simulink model "PassVeh14DOF"  (R2026b)
settings: Solver=ode23tb  StopTime=inf  FixedStep=.001  RelTol=1e-1  EnableMultiTasking=on
model workspace (MAT data in the model file):
  AlgnTrqCambCompl = [0 0 0 0]
  AlgnTrqSteerCompl = [0 0 0 0]
  AxlIxx = 62.3745166667
  AxlM = 160
  BumpCamber = [0 0 0 0]
  BumpCaster = [0 0 0 0]
  BumpSteer = [0 0 0 0]
  CambVsSteerAng = [0 0 0 0]
  CastVsSteerAng = [0 0 0 0]
  Cps = 2
  Cz = 5565.2246438
  CzWhlAxl = 11490.971257
  DCT_Param : object (value not decoded)
  Downshift_Speeds = [9.5625 12.9375 16.3125 19.6875 23.0625 26.4375 29.8125 33.1875 36.5625 39.9375 43.3125 46.6875 ... (28 elements, 4x7)]
  F0z = [2886 2907]
  F0zWhlAxl = 2907
  Hmax = 0.25
  Kz = 52451.0065793
  KzWhlAxl = 138031.612078
  LatCambCompl = [0 0 0 0]
  LatSteerCompl = [0 0 0 0]
  LatWhlCtrComplLat = [0 0 0 0]
  LatWhlCtrComplLng = [0  0  0  0; 0  0  0  0]
  LatWhlCtrDisp = [0 0 0 0]
  LngCambCompl = [0  0  0  0; 0  0  0  0]
  LngCastCompl = [0  0  0  0; 0  0  0  0]
  LngSteerCompl = [0  0  0  0; 0  0  0  0]
  LngWhlCtrCompl = [0  0  0  0; 0  0  0  0]
  LngWhlCtrDisp = [0 0 0 0]
  MotRatios = [1 1]
  NCyl = 6
  NrmlWhlFrcOff = [2886 2886 2907 2907]
  NrmlWhlRates = [52.4510065793 52.4510065793 52.4510065793 52.4510065793]
  Pedal_Positions = [0.1 0.4 0.5 0.9]
  Pstd = 101325
  Rair = 287
  RollCamber : object (value not decoded)
  RollCaster : object (value not decoded)
  RollSteer : object (value not decoded)
  RollStiffArb = [0 0]
  RollStiffArbFrnt = 800
  RollStiffNoArb = [0 0]
  RollStiffNoArbFrnt = 0
  RollStiffNoTwstRear = 0
  ShckFrcVsCompRate = [5.5652246438 5.5652246438 5.5652246438 5.5652246438]
  StatCamber = [0 0 0 0]
  StatCaster = [0 0 0 0]
  StatLdWhlR = [0.3 0.3 0.3 0.3]
  StatToe = [0 0 0 0]
  Trans : object (value not decoded)
  Tstd = 293.15
  Upshift_Speeds = [12.9375 16.3125 19.6875 33 26.4375 29.8125 33.1875 52.5 39.9375 43.3125 46.6875 77.25 ... (28 elements, 4x7)]
  VEH : object (value not decoded)
  Vd = 0.00346
  VrtLdTrnsfr = [0 0 0 0]
  WH : Mass (value not decoded)
  dt3D = 0.05
  f_air = [0 0 0 0 0 0 0 0 0 0 0 0 ... (256 elements, 16x16)]
  f_co = [0 0 0 0 0 0 0 0 0 0 0 0 ... (256 elements, 16x16)]
  f_co2 = [0 0 0 0 0 0 0 0 0 0 0 0 ... (256 elements, 16x16)]
  f_eff = [352.135682859 352.135682859 320.724378192 303.655312657 295.930136708 291.240087194 291.240271258 291.240312459 291.240275452 291.240198499 291.240100781 291.240018769 ... (256 elements, 16x16)]
  f_fuel = [0 0 0 0 0 0 0 0 0 0 0 0 ... (256 elements, 16x16)]
  f_hc = [0 0 0 0 0 0 0 0 0 0 0 0 ... (256 elements, 16x16)]
  f_nox = [0 0 0 0 0 0 0 0 0 0 0 0 ... (256 elements, 16x16)]
  f_pm = [0 0 0 0 0 0 0 0 0 0 0 0 ... (256 elements, 16x16)]
  f_susp_axl_bp = [1 2]
  f_susp_dz_bp = [-0.325022776267 -0.315022776267 -0.305022776267 -0.205022776267 -0.105022776267 -0.00502277626717 0.0949772237328 0.194977223733 0.204977223733 0.214977223733]
  f_susp_dzdot_bp = [-3 -0.3 -0.2 -0.1 0 0.1 0.2 0.3 3]
  f_susp_fmz = [-144070.391448 -93629.24037 -75929.1118915 -20630.5828179 -15385.48216 -10140.3815021 -4895.28084414 349.819813785 -31916.3973792 18437.6709544 -83996.1993354 -33555.0482577 ... (43920 elements, 10x9x61x2x4)]
  f_susp_geom = [0 0 0 0 0 0 0 0 0 0 0 0 ... (3660 elements, 10x61x2x3)]
  f_susp_strgdelta_bp = [-0.523598775598 -0.506145483078 -0.488692190558 -0.471238898038 -0.453785605519 -0.436332312999 -0.418879020479 -0.401425727959 -0.383972435439 -0.366519142919 -0.349065850399 -0.331612557879 ... (61 elements, 1x61)]
  f_tbrake = [0 76.8593923996 105.140482948 131.533638111 157.926793274 176.658631717 176.65727296 176.656856686 176.656879077 176.657093756 176.657404516 176.65772406 ... (256 elements, 16x16)]
  f_tbrake_n_bpt = [0 649.519052838 912.419621844 1175.32019085 1438.22075986 1701.12132886 1964.02189787 2226.92246687 2489.82303588 2752.72360489 3015.62417389 3278.5247429 ... (16 elements, 1x16)]
  f_tbrake_t_bpt = [0 34.6410161514 61.0341713143 87.4273264773 113.82048164 140.213636803 166.606791966 192.999947129 219.393102292 245.786257455 272.179412618 298.572567781 ... (16 elements, 1x16)]
  f_texh = [766.752464599 766.752464599 786.17542386 801.679939032 884.591982581 910.574397722 910.571871054 910.570774534 910.570601632 910.570821151 910.571247242 910.571639815 ... (256 elements, 16x16)]
  f_twc_eff_co = [0.17 0.25 0.45 0.99 0.99 0.99 0.99]
  f_twc_eff_hc = [0.21 0.375 0.75 0.98 0.98 0.98 0.98]
  f_twc_eff_lam = [0.909090909 0.944055944 0.979020979 1 1.013986014 1.048951049 1.083916084]
  f_twc_eff_nox = [0.98 0.98 0.98 0.97 0.05 0.02 0]
  numWheel = 4
symbols that are objects in the model workspace (value not decoded): VEH
libraries: vehdynlibtire x12, vehdynlibsuspension x8, autolibutils x5, sharedtransform x5, shared6dof x2, vehdynlibeom x1, vehdynlibtirecommon x1, matrix_library x1
(part 8 of 9)

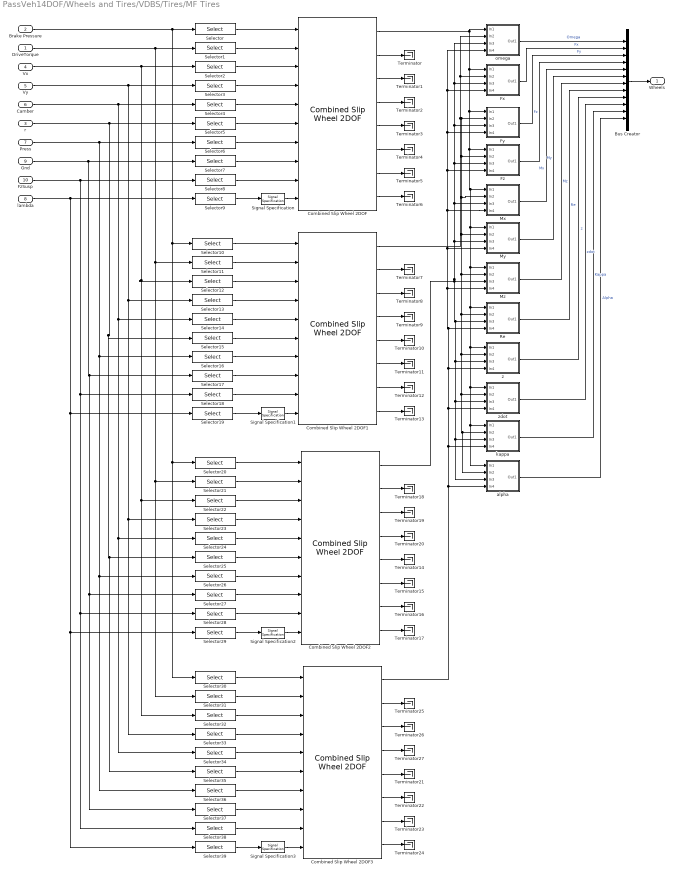
== system PassVeh14DOF/Wheels and Tires/VDBS/Tires/MF Tires ==
  DriveTorque : Inport
  Brake Pressure : Inport  Port=2
  r : Inport  Port=3
  Vx : Inport  Port=4
  Vy : Inport  Port=5
  Camber : Inport  Port=6
  Press : Inport  Port=7  Unit=Pa
  lambda : Inport  Port=8  Unit=1
  Gnd : Inport  Port=9
  FzSusp : Inport  Port=10
  Bus Creator : BusCreator  Inputs=12
  Combined Slip Wheel 2DOF{,1..3} (4 alike) : vehdynlibtire/Combined Slip Wheel 2DOF  tireType=Mid-size passenger car 235/45R18  tireParamSet=vdynPassCar.mat  scaleFactorInput=on  vertType=Magic Formula  plySteer=off  turnslip=off  BrakeType=Disc  mu_static=.3  mu_kinetic=.2  drum_abore=0.0508  drum_a=0.123  drum_c=0.212  drum_r=0.15  drum_theta1=0  drum_theta2=126  disk_abore=.05  Rm=.177  num_pads=2  brake_p_bpt=[1 11.4736842105263 21.9473684210526 32.4210526315789 42.8947368421053 53.3684210526316 63.8421052631579 74.3157894736842 84.7894736842105 95.2631578947368 105.736842105263 116.210526315789 126.684210526316 137.157894736842 147.631578947368 158.105263157895 168.578947368421 179.052631578947 189.526315789474 200]  brake_n_bpt=[0 52.6315789473684 105.263157894737 157.894736842105 210.526315789474 263.157894736842 315.789473684211 368.421052631579 421.052631578947 473.684210526316 526.315789473684 578.947368421053 631.578947368421 684.210526315789 736.842105263158 789.473684210526 842.105263157895 894.736842105263 947.368421052632 1000]  f_brake_t=[43.4900602404453 42.5056030554862 41.5350898940194 40.5780454442085 39.6340111501808 38.7025443887544 37.7832176914519 36.8756180088306 35.9793460143796 35.0940154454303 34.2192524787115 33.3546951383474 32.4999927342521 31.6548053290159 30.8188032315107 29.991666515561 29.1730845621415 28.362755623661 27.5603864089927 26.765691687993;498.991217495636 487.695866636631 476.560505099801 465.579679307235 454.748127933653 444.060772460445 433.51270824929 423.099196101319 412.81565427025 402.657650900201 392.620896861006 382.701238955775 372.894653477208 363.197240090814 353.605216024701 344.114910546964 334.722759712992 325.425301366216 316.219170376863 307.10109410434;954.492374750826 932.886130217776 911.585920305583 890.581313170261 869.862244717126 849.419000532136 829.242198807128 809.322774193808 789.651962526121 770.221286354971 751.0225412433 732.047782773203 713.289314220164 694.739674852612 676.391628817892 658.238154578366 640.272434863842 622.48784710877 604.877954344734 587.436496520688;1409.99353200602 1378.07639379892 1346.61133551136 1315.58294703329 1284.9763615006 1254.77722860383 1224.97168936497 1195.5463522863 1166.48827078199 1137.78492180974 1109.42418562559 1081.39432659063 1053.68397496312 1026.28210961441 999.178041611083 972.361398609768 945.822110014692 919.550392851325 893.536738312604 867.771898937035;1865.49468926121 1823.26665738007 1781.63675071715 1740.58458089631 1700.09047828407 1660.13545667552 1620.7011799228 1581.76993037878 1543.32457903786 1505.34855726451 1467.82583000789 1430.74087040806 1394.07863570608 1357.82454437621 1321.96445440427 1286.48464264117 1251.37178516554 1216.61293859388 1182.19552228048 1148.10730135338;2320.9958465164 2268.45692096121 2216.66216592293 2165.58621475934 2115.20459506754 2065.49368474721 2016.43067048064 1967.99350847127 1920.16088729373 1872.91219271928 1826.22747439018 1780.08741422549 1734.47329644903 1689.36697913801 1644.75086719747 1600.60788667257 1556.92146031639 1513.67548433643 1470.85430624835 1428.44270376973;2776.49700377159 2713.64718454235 2651.68758112871 2590.58784862237 2530.31871185102 2470.8519128189 2412.16016103848 2354.21708656376 2296.9971955496 2240.47582817405 2184.62911877248 2129.43395804292 2074.86795719199 2020.9094138998 1967.53727999066 1914.73113070398 1862.47113546724 1810.73803007899 1759.51309021622 1708.77810618608;3231.99816102678 3158.8374481235 3086.71299633449 3015.58948248539 2945.43282863449 2876.21014089059 2807.88965159632 2740.44066465625 2673.83350380547 2608.03946362882 2543.03076315477 2478.78050186034 2415.26261793494 2352.4518486616 2290.32369278385 2228.85437473538 2168.02081061809 2107.80057582154 2048.17187418409 1989.11350860242;3687.49931828197 3604.02771170464 3521.73841154027 3440.59111634842 3360.54694541796 3281.56836896228 3203.61914215416 3126.66424274874 3050.66981206134 2975.60309908359 2901.43240753707 2828.12704567777 2755.6572786779 2683.9942834234 2613.11010557704 2542.97761876678 2473.57048576894 2404.8631215641 2336.83065815196 2269.44891101877;4143.00047553716 4049.21797528579 3956.76382674606 3865.59275021144 3775.66106220143 3686.92659703397 3599.34863271199 3512.88782084123 3427.50612031721 3343.16673453836 3259.83405191936 3177.4735894952 3096.05193942085 3015.5367181852 2935.89651837023 2857.10086279818 2779.12016091979 2701.92566730665 2625.48944211983 2549.78431343512;4598.50163279235 4494.40823886693 4391.78924195184 4290.59438407447 4190.77517898491 4092.28482510566 3995.07812326983 3899.11139893372 3804.34242857308 3710.73036999313 3618.23569630166 3526.82013331263 3436.44660016381 3347.079152947 3258.68293116342 3171.22410682959 3084.66983607064 2998.98821304921 2914.1482260877 2830.11971585147;5054.00279004754 4939.59850244808 4826.81465715762 4715.59601793749 4605.88929576838 4497.64305317735 4390.80761382767 4285.3349770262 4181.17873682896 4078.2940054479 3976.63734068395 3876.16667713006 3776.84126090677 3678.62158770879 3581.46934395661 3485.34735086099 ...(+2764 chars)]  NOMPRES=262000  PRESMAX=1000000  PRESMIN=10000  FNOMIN=4300  FZMAX=8600  FZMIN=100  VXLOW=1  KPUMAX=1.5  KPUMIN=-1.5  ALPMAX=1.5  ALPMIN=-1.5  CAMMAX=0.17453  CAMMIN=-0.17453  LONGVL=16.7  FxRelFreqLwrLim=200*pi  FyRelFreqLwrLim=0  MyRelFreqLwrLim=50*pi  omegao=0  UNLOADED_RADIUS=0.33454  WIDTH=0.235  RIM_RADIUS=0.2286  ASPECT_RATIO=0.45  MASS=11.2  IYY=1.084  br=1e-3  GRAVITY=-9.81  LFZO=1  LMUX=1  LMUY=1  LMUV=0  LKX=1  LKY=1  LCX=1  LCY=1  LEX=1  LEY=1  LHX=1  LHY=1  LVX=1  LVY=1  LKYC=1  LKZC=1  LTR=1  LRES=1  LXAL=1  LYKA=1  LVYKA=1  LS=1  LCZ=1  LMX=1  LVMX=1  LMY=1  LMP=1  zo=.015+VEH.InitialVertPosition  zdoto=0  BREFF=8.25094594147963  DREFF=0.260468730454265  FREFF=0.0735298544471851  Q_RE0=1.00866439868088  Q_V1=0.000760413786224011  Q_V2=0.0463384792019201  Q_FZ1=0  Q_FZ2=15.6870832810226  Q_FZ3=0  Q_FCX=0.138643970247602  Q_FCY=0.10843499565426  Q_FCY2=-0.465763352339538  PFZ1=0.69958166705601  VERTICAL_STIFFNESS=207885.061134007  VERTICAL_DAMPING=500  BOTTOM_OFFST=0.00990653336182505  BOTTOM_STIFF=1999075.87051971  Q_CAM1=0  Q_CAM2=0  Q_CAM3=0  Q_FYS1=0  Q_FYS2=0  Q_FYS3=0  LONGITUDINAL_STIFFNESS=388714.175879854  LATERAL_STIFFNESS=157087.404633332  PCFX1=0.18539229191199  PCFX2=0  PCFX3=0  PCFY1=0.163183345037677  PCFY2=0  PCFY3=0.249094918231954  Q_RA1=0.675942571700787  Q_RA2=0.73800463546164  Q_RB1=1.04487486456705  Q_RB2=-1.191763806629  PCX1=1.58523057950359  PDX1=1.0239116238178  PDX2=-0.0842405110022724  PDX3=0  PEX1=0.110312777158455  PEX2=0.313468516038146  PEX3=0  PEX4=0.0016060905760045  PKX1=21.3872544684023  PKX2=14.0006541873175  PKX3=-0.405326109653452  PHX1=0.000212599305364818  PHX2=0.00115950515263055  PVX1=1.59236164471432e-05  PVX2=0.000104321112127671  PPX1=-0.349461321276586  PPX2=0.387840040616429  PPX3=-0.0969947336569324  PPX4=0.0632271859795801  RBX1=12.7633329850276  RBX2=9.5787123658471  RBX3=0  RCX1=1.02796280922059  REX1=-0.45202516851367  REX2=-0.47304886171176  RHX1=0.000233272373115809  QSX1=-0.00788307788961443  QSX2=0.954629515459396  QSX3=0.0155855777667025  QSX4=0.125904607142414  QSX5=1.01110069703963  QSX6=20.1938577118433  QSX7=0.310818120717083  QSX8=-0.0430823751139655  QSX9=0.636494404888216  QSX10=0.142438060591663  QSX11=0.346766530036373  QSX12=0  QSX13=0  QSX14=0  PPMX1=0  PCY1=1.34299950037631  PDY1=0.878267729082195  PDY2=-0.0644597923147385  PDY3=0  PEY1=-0.809776534470972  PEY2=-0.600180598867198  PEY3=0.0991732552633487  PEY4=-6.5577974035573  PEY5=0  PKY1=-15.5714726518315  PKY2=1.73126522291751  PKY3=0.365349873517229  PKY4=1.98176755955416  PKY5=0  PKY6=-0.884005199550313  PKY7=-0.237259727611847  PHY1=-0.00183370557235628  PHY2=0.00346401302716671  PVY1=-0.00675427560163264  PVY2=0.036379218103843  PVY3=-0.163543984089166  PVY4=-0.491003349625726  PPY1=-0.62059646553185  PPY2=-0.0647824842338686  PPY3=-0.164648843290686  PPY4=0.283193909060098  PPY5=0  RBY1=10.7588809173639  RBY2=7.70420065295029  RBY3=3.40283755070691e-06  RBY4=0  RCY1=1.06691874059059  REY1=0.308244924574305  REY2=7.48775032604508e-06  RHY1=0.0118479204960415  RHY2=7.63650177161071e-06  RVY1=0.0560024425050078  RVY2=7.48487127056197e-06  RVY3=0  RVY4=98.4047026517149  RVY5=2.02759273900054  RVY6=15.7623064923347  QSY1=0.00699077564863536  QSY2=0  QSY3=0.00153535478298811  QSY4=8.55710322455322e-05  QSY5=0  QSY6=0  QSY7=0.89443879773793  QSY8=-0.403227641260894  QBZ1=11.666656027484  QBZ2=-1.30355438574485  QBZ3=0  QBZ4=0.177918305399071  QBZ5=-0.162481135068033  QBZ6=0  QBZ9=30.1445534682089  QBZ10=0  QCZ1=1.29026978207574  QDZ1=0.0886972644991399  QDZ2=-0.0058634820161856  QDZ3=0.3805597481383  QDZ4=0  QDZ6=0.00160914918118959  QDZ7=-0.00211036330862154  QDZ8=-0.13921904912557  QDZ9=0.00816585550028243  QDZ10=0  QDZ11=0  QEZ1=-2.19802254534746  QEZ2=1.01850535789165  QEZ3=0  QEZ4=0.278379679112054  QEZ5=-0.548414722765386  QHZ1=0.00148361198869669  QHZ2=0.00202017567585904  QHZ3=0.240316641332066  QHZ4=-0.210114035738085  PPZ1=-0.443927982388615  PPZ2=0  SSZ1=0.00914999585397887  SSZ2=0.0389830656052735  SSZ3=0  SSZ4=0  PDXP1=0.396718274678791  PDXP2=0  PDXP3=0  PKYP1=1.00587060633573  PDYP1=0.40483048923438  PDYP2=0  PDYP3=0  PDYP4=0  PHYP1=0.992731942067188  PHYP2=0.150352945499914  PHYP3=0  PHYP4=-3.98988682633674  PECP1=0.502379254513503  PECP2=0  QDTP1=10.0178654287947  QCRP1=0.200627747200702  QCRP2=0.0995735881599772  QBRP1=0.0997107127960717  QDRP1=1.01432910167423  QDRP2=0  aMode=2
  Fx : Subsystem
  Fy : Subsystem
  Fz : Subsystem
  Mx : Subsystem
  My : Subsystem
  Mz : Subsystem
  Re : Subsystem
  Selector{,1..8} (9 alike) : Selector  InputPortWidth=4  IndexOptions=Index vector (dialog)  Indices=1  OutputSizes=1
  Selector{10..18} (9 alike) : Selector  InputPortWidth=4  IndexOptions=Index vector (dialog)  Indices=2  OutputSizes=1
  Selector19 : Selector  NumberOfDimensions=2  InputPortWidth=4  IndexOptions=Select all,Index vector (dialog)  Indices=1,2  OutputSizes=1,1
  Selector{20..28} (9 alike) : Selector  InputPortWidth=4  IndexOptions=Index vector (dialog)  Indices=3  OutputSizes=1
  Selector29 : Selector  NumberOfDimensions=2  InputPortWidth=4  IndexOptions=Select all,Index vector (dialog)  Indices=1,3  OutputSizes=1,1
  Selector{30..38} (9 alike) : Selector  InputPortWidth=4  IndexOptions=Index vector (dialog)  Indices=4  OutputSizes=1
  Selector39 : Selector  NumberOfDimensions=2  InputPortWidth=4  IndexOptions=Select all,Index vector (dialog)  Indices=1,4  OutputSizes=1,1
  Selector9 : Selector  NumberOfDimensions=2  InputPortWidth=4  IndexOptions=Select all,Index vector (dialog)  Indices=1,1  OutputSizes=1,1
  Signal Specification{,1..3} (4 alike) : SignalSpecification  Unit=1
  Terminator{,1..27} (28 alike) : Terminator
  alpha : Subsystem
  kappa : Subsystem
  omega : Subsystem
  z : Subsystem
  zdot : Subsystem
  Wheels : Outport  VectorParamsAs1DForOutWhenUnconnected=off
  wires:
  Bus Creator/1 -> Wheels/1
  Brake Pressure/1 -> Selector30/1, Selector20/1, Selector10/1, Selector/1
  DriveTorque/1 -> Selector31/1, Selector21/1, Selector11/1, Selector1/1
  Vx/1 -> Selector12/1, Selector32/1, Selector22/1, Selector2/1
  Selector/1 -> Combined Slip Wheel 2DOF/1
  Selector1/1 -> Combined Slip Wheel 2DOF/2
  Selector7/1 -> Combined Slip Wheel 2DOF/8
  Selector6/1 -> Combined Slip Wheel 2DOF/7
  Selector5/1 -> Combined Slip Wheel 2DOF/6
  Selector4/1 -> Combined Slip Wheel 2DOF/5
  Selector9/1 -> Signal Specification/1
  Selector8/1 -> Combined Slip Wheel 2DOF/9
  Camber/1 -> Selector34/1, Selector24/1, Selector14/1, Selector4/1
  Vy/1 -> Selector33/1, Selector23/1, Selector13/1, Selector3/1
  r/1 -> Selector15/1, Selector35/1, Selector25/1, Selector5/1
  Press/1 -> Selector36/1, Selector26/1, Selector16/1, Selector6/1
  Gnd/1 -> Selector37/1, Selector27/1, Selector17/1, Selector7/1
  FzSusp/1 -> Selector38/1, Selector28/1, Selector18/1, Selector8/1
  lambda/1 -> Selector9/1, Selector19/1, Selector39/1, Selector29/1
  Selector18/1 -> Combined Slip Wheel 2DOF1/9
  Selector19/1 -> Signal Specification1/1
  Selector14/1 -> Combined Slip Wheel 2DOF1/5
  Selector15/1 -> Combined Slip Wheel 2DOF1/6
  Selector16/1 -> Combined Slip Wheel 2DOF1/7
  Selector17/1 -> Combined Slip Wheel 2DOF1/8
  Selector12/1 -> Combined Slip Wheel 2DOF1/3
  Selector13/1 -> Combined Slip Wheel 2DOF1/4
  Selector11/1 -> Combined Slip Wheel 2DOF1/2
  Selector10/1 -> Combined Slip Wheel 2DOF1/1
  Selector30/1 -> Combined Slip Wheel 2DOF3/1
  Selector31/1 -> Combined Slip Wheel 2DOF3/2
  Selector33/1 -> Combined Slip Wheel 2DOF3/4
  Selector32/1 -> Combined Slip Wheel 2DOF3/3
  Selector37/1 -> Combined Slip Wheel 2DOF3/8
  Selector36/1 -> Combined Slip Wheel 2DOF3/7
  Selector35/1 -> Combined Slip Wheel 2DOF3/6
  Selector34/1 -> Combined Slip Wheel 2DOF3/5
  Selector39/1 -> Signal Specification3/1
  Selector38/1 -> Combined Slip Wheel 2DOF3/9
  Selector28/1 -> Combined Slip Wheel 2DOF2/9
  Selector29/1 -> Signal Specification2/1
  Selector24/1 -> Combined Slip Wheel 2DOF2/5
  Selector25/1 -> Combined Slip Wheel 2DOF2/6
  Selector26/1 -> Combined Slip Wheel 2DOF2/7
  Selector27/1 -> Combined Slip Wheel 2DOF2/8
  Selector22/1 -> Combined Slip Wheel 2DOF2/3
  Selector23/1 -> Combined Slip Wheel 2DOF2/4
  Selector21/1 -> Combined Slip Wheel 2DOF2/2
  Selector20/1 -> Combined Slip Wheel 2DOF2/1
  Combined Slip Wheel 2DOF1/1 -> omega/2(In2), Fx/2(In2), Mx/2(In2), My/2(In2), alpha/2(In2), kappa/2(In2), zdot/2(In2), z/2(In2), Re/2(In2), Mz/2(In2), Fz/2(In2), Fy/2(In2)
  Combined Slip Wheel 2DOF2/1 -> omega/3(In3), Fx/3(In3), Fy/3(In3), Fz/3(In3), Mx/3(In3), My/3(In3), alpha/3(In3), kappa/3(In3), zdot/3(In3), z/3(In3), Re/3(In3), Mz/3(In3)
  Combined Slip Wheel 2DOF3/1 -> omega/4(In4), Fx/4(In4), Fy/4(In4), Fz/4(In4), Mx/4(In4), My/4(In4), Mz/4(In4), Re/4(In4), z/4(In4), zdot/4(In4), kappa/4(In4), alpha/4(In4)
  Combined Slip Wheel 2DOF/1 -> omega/1(In1), Mx/1(In1), My/1(In1), alpha/1(In1), kappa/1(In1), zdot/1(In1), z/1(In1), Re/1(In1), Mz/1(In1), Fz/1(In1), Fy/1(In1), Fx/1(In1)
  omega/1(Out1) -> Bus Creator/1  "Omega"
  Fx/1(Out1) -> Bus Creator/2  "Fx"
  Mz/1(Out1) -> Bus Creator/7  "Mz"
  Fz/1(Out1) -> Bus Creator/4  "Fz"
  Re/1(Out1) -> Bus Creator/8  "Re"
  z/1(Out1) -> Bus Creator/9  "z"
  zdot/1(Out1) -> Bus Creator/10  "zdot"
  Mx/1(Out1) -> Bus Creator/5  "Mx"
  My/1(Out1) -> Bus Creator/6  "My"
  kappa/1(Out1) -> Bus Creator/11  "Kappa"
  Fy/1(Out1) -> Bus Creator/3  "Fy"
  Selector2/1 -> Combined Slip Wheel 2DOF/3
  Selector3/1 -> Combined Slip Wheel 2DOF/4
  Signal Specification/1 -> Combined Slip Wheel 2DOF/10
  Signal Specification1/1 -> Combined Slip Wheel 2DOF1/10
  Signal Specification2/1 -> Combined Slip Wheel 2DOF2/10
  Signal Specification3/1 -> Combined Slip Wheel 2DOF3/10
  Combined Slip Wheel 2DOF/2 -> Terminator/1
  Combined Slip Wheel 2DOF/3 -> Terminator1/1
  Combined Slip Wheel 2DOF/4 -> Terminator2/1
  Combined Slip Wheel 2DOF/7 -> Terminator5/1
  Combined Slip Wheel 2DOF/6 -> Terminator4/1
  Combined Slip Wheel 2DOF/5 -> Terminator3/1
  Combined Slip Wheel 2DOF/8 -> Terminator6/1
  Combined Slip Wheel 2DOF1/2 -> Terminator7/1
  Combined Slip Wheel 2DOF1/3 -> Terminator8/1
  Combined Slip Wheel 2DOF1/4 -> Terminator9/1
  Combined Slip Wheel 2DOF1/5 -> Terminator10/1
  Combined Slip Wheel 2DOF1/6 -> Terminator11/1
  Combined Slip Wheel 2DOF1/7 -> Terminator12/1
  Combined Slip Wheel 2DOF1/8 -> Terminator13/1
  Combined Slip Wheel 2DOF2/2 -> Terminator18/1
  Combined Slip Wheel 2DOF2/3 -> Terminator19/1
  Combined Slip Wheel 2DOF2/4 -> Terminator20/1
  Combined Slip Wheel 2DOF2/5 -> Terminator14/1
  Combined Slip Wheel 2DOF2/6 -> Terminator15/1
  Combined Slip Wheel 2DOF2/7 -> Terminator16/1
  Combined Slip Wheel 2DOF2/8 -> Terminator17/1
  Combined Slip Wheel 2DOF3/2 -> Terminator25/1
  Combined Slip Wheel 2DOF3/3 -> Terminator26/1
  Combined Slip Wheel 2DOF3/4 -> Terminator27/1
  Combined Slip Wheel 2DOF3/5 -> Terminator21/1
  Combined Slip Wheel 2DOF3/6 -> Terminator22/1
  Combined Slip Wheel 2DOF3/7 -> Terminator23/1
  Combined Slip Wheel 2DOF3/8 -> Terminator24/1
  alpha/1(Out1) -> Bus Creator/12  "Alpha"

== system PassVeh14DOF/Wheels and Tires/VDBS/Tires/MF Tires Vector ==
  DriveTorque : Inport
  Brake Pressure : Inport  Port=2
  r : Inport  Port=3
  Vx : Inport  Port=4
  Vy : Inport  Port=5
  Camber : Inport  Port=6
  Press : Inport  Port=7  Unit=Pa
  lambda : Inport  Port=8  Unit=1
  Gnd : Inport  Port=9
  FzSusp : Inport  Port=10
  Combined Slip Wheel 2DOF : vehdynlibtire/Combined Slip Wheel 2DOF  tireType=Mid-size passenger car 235/45R18  tireParamSet=vdynPassCar.mat  scaleFactorInput=on  vertType=Magic Formula  plySteer=off  turnslip=off  BrakeType=Disc  mu_static=.3  mu_kinetic=.2  drum_abore=0.0508  drum_a=0.123  drum_c=0.212  drum_r=0.15  drum_theta1=0  drum_theta2=126  disk_abore=.05  Rm=.177  num_pads=2  brake_p_bpt=[1 11.4736842105263 21.9473684210526 32.4210526315789 42.8947368421053 53.3684210526316 63.8421052631579 74.3157894736842 84.7894736842105 95.2631578947368 105.736842105263 116.210526315789 126.684210526316 137.157894736842 147.631578947368 158.105263157895 168.578947368421 179.052631578947 189.526315789474 200]  brake_n_bpt=[0 52.6315789473684 105.263157894737 157.894736842105 210.526315789474 263.157894736842 315.789473684211 368.421052631579 421.052631578947 473.684210526316 526.315789473684 578.947368421053 631.578947368421 684.210526315789 736.842105263158 789.473684210526 842.105263157895 894.736842105263 947.368421052632 1000]  f_brake_t=[43.4900602404453 42.5056030554862 41.5350898940194 40.5780454442085 39.6340111501808 38.7025443887544 37.7832176914519 36.8756180088306 35.9793460143796 35.0940154454303 34.2192524787115 33.3546951383474 32.4999927342521 31.6548053290159 30.8188032315107 29.991666515561 29.1730845621415 28.362755623661 27.5603864089927 26.765691687993;498.991217495636 487.695866636631 476.560505099801 465.579679307235 454.748127933653 444.060772460445 433.51270824929 423.099196101319 412.81565427025 402.657650900201 392.620896861006 382.701238955775 372.894653477208 363.197240090814 353.605216024701 344.114910546964 334.722759712992 325.425301366216 316.219170376863 307.10109410434;954.492374750826 932.886130217776 911.585920305583 890.581313170261 869.862244717126 849.419000532136 829.242198807128 809.322774193808 789.651962526121 770.221286354971 751.0225412433 732.047782773203 713.289314220164 694.739674852612 676.391628817892 658.238154578366 640.272434863842 622.48784710877 604.877954344734 587.436496520688;1409.99353200602 1378.07639379892 1346.61133551136 1315.58294703329 1284.9763615006 1254.77722860383 1224.97168936497 1195.5463522863 1166.48827078199 1137.78492180974 1109.42418562559 1081.39432659063 1053.68397496312 1026.28210961441 999.178041611083 972.361398609768 945.822110014692 919.550392851325 893.536738312604 867.771898937035;1865.49468926121 1823.26665738007 1781.63675071715 1740.58458089631 1700.09047828407 1660.13545667552 1620.7011799228 1581.76993037878 1543.32457903786 1505.34855726451 1467.82583000789 1430.74087040806 1394.07863570608 1357.82454437621 1321.96445440427 1286.48464264117 1251.37178516554 1216.61293859388 1182.19552228048 1148.10730135338;2320.9958465164 2268.45692096121 2216.66216592293 2165.58621475934 2115.20459506754 2065.49368474721 2016.43067048064 1967.99350847127 1920.16088729373 1872.91219271928 1826.22747439018 1780.08741422549 1734.47329644903 1689.36697913801 1644.75086719747 1600.60788667257 1556.92146031639 1513.67548433643 1470.85430624835 1428.44270376973;2776.49700377159 2713.64718454235 2651.68758112871 2590.58784862237 2530.31871185102 2470.8519128189 2412.16016103848 2354.21708656376 2296.9971955496 2240.47582817405 2184.62911877248 2129.43395804292 2074.86795719199 2020.9094138998 1967.53727999066 1914.73113070398 1862.47113546724 1810.73803007899 1759.51309021622 1708.77810618608;3231.99816102678 3158.8374481235 3086.71299633449 3015.58948248539 2945.43282863449 2876.21014089059 2807.88965159632 2740.44066465625 2673.83350380547 2608.03946362882 2543.03076315477 2478.78050186034 2415.26261793494 2352.4518486616 2290.32369278385 2228.85437473538 2168.02081061809 2107.80057582154 2048.17187418409 1989.11350860242;3687.49931828197 3604.02771170464 3521.73841154027 3440.59111634842 3360.54694541796 3281.56836896228 3203.61914215416 3126.66424274874 3050.66981206134 2975.60309908359 2901.43240753707 2828.12704567777 2755.6572786779 2683.9942834234 2613.11010557704 2542.97761876678 2473.57048576894 2404.8631215641 2336.83065815196 2269.44891101877;4143.00047553716 4049.21797528579 3956.76382674606 3865.59275021144 3775.66106220143 3686.92659703397 3599.34863271199 3512.88782084123 3427.50612031721 3343.16673453836 3259.83405191936 3177.4735894952 3096.05193942085 3015.5367181852 2935.89651837023 2857.10086279818 2779.12016091979 2701.92566730665 2625.48944211983 2549.78431343512;4598.50163279235 4494.40823886693 4391.78924195184 4290.59438407447 4190.77517898491 4092.28482510566 3995.07812326983 3899.11139893372 3804.34242857308 3710.73036999313 3618.23569630166 3526.82013331263 3436.44660016381 3347.079152947 3258.68293116342 3171.22410682959 3084.66983607064 2998.98821304921 2914.1482260877 2830.11971585147;5054.00279004754 4939.59850244808 4826.81465715762 4715.59601793749 4605.88929576838 4497.64305317735 4390.80761382767 4285.3349770262 4181.17873682896 4078.2940054479 3976.63734068395 3876.16667713006 3776.84126090677 3678.62158770879 3581.46934395661 3485.34735086099 ...(+2764 chars)]  NOMPRES=262000  PRESMAX=1000000  PRESMIN=10000  FNOMIN=4300  FZMAX=8600  FZMIN=100  VXLOW=1  KPUMAX=1.5  KPUMIN=-1.5  ALPMAX=1.5  ALPMIN=-1.5  CAMMAX=0.17453  CAMMIN=-0.17453  LONGVL=16.7  FxRelFreqLwrLim=40*pi  FyRelFreqLwrLim=0  MyRelFreqLwrLim=40*pi  omegao=0  UNLOADED_RADIUS=0.33454  WIDTH=0.235  RIM_RADIUS=0.2286  ASPECT_RATIO=0.45  MASS=11.2  IYY=1.084  br=1e-3  GRAVITY=-9.81  LFZO=1  LMUX=1  LMUY=1  LMUV=0  LKX=1  LKY=1  LCX=1  LCY=1  LEX=1  LEY=1  LHX=1  LHY=1  LVX=1  LVY=1  LKYC=1  LKZC=1  LTR=1  LRES=1  LXAL=1  LYKA=1  LVYKA=1  LS=1  LCZ=1  LMX=1  LVMX=1  LMY=1  LMP=1  zo=.015+VEH.InitialVertPosition  zdoto=0  BREFF=8.25094594147963  DREFF=0.260468730454265  FREFF=0.0735298544471851  Q_RE0=1.00866439868088  Q_V1=0.000760413786224011  Q_V2=0.0463384792019201  Q_FZ1=0  Q_FZ2=15.6870832810226  Q_FZ3=0  Q_FCX=0.138643970247602  Q_FCY=0.10843499565426  Q_FCY2=-0.465763352339538  PFZ1=0.69958166705601  VERTICAL_STIFFNESS=207885.061134007  VERTICAL_DAMPING=500  BOTTOM_OFFST=0.00990653336182505  BOTTOM_STIFF=1999075.87051971  Q_CAM1=0  Q_CAM2=0  Q_CAM3=0  Q_FYS1=0  Q_FYS2=0  Q_FYS3=0  LONGITUDINAL_STIFFNESS=388714.175879854  LATERAL_STIFFNESS=157087.404633332  PCFX1=0.18539229191199  PCFX2=0  PCFX3=0  PCFY1=0.163183345037677  PCFY2=0  PCFY3=0.249094918231954  Q_RA1=0.675942571700787  Q_RA2=0.73800463546164  Q_RB1=1.04487486456705  Q_RB2=-1.191763806629  PCX1=1.58523057950359  PDX1=1.0239116238178  PDX2=-0.0842405110022724  PDX3=0  PEX1=0.110312777158455  PEX2=0.313468516038146  PEX3=0  PEX4=0.0016060905760045  PKX1=21.3872544684023  PKX2=14.0006541873175  PKX3=-0.405326109653452  PHX1=0.000212599305364818  PHX2=0.00115950515263055  PVX1=1.59236164471432e-05  PVX2=0.000104321112127671  PPX1=-0.349461321276586  PPX2=0.387840040616429  PPX3=-0.0969947336569324  PPX4=0.0632271859795801  RBX1=12.7633329850276  RBX2=9.5787123658471  RBX3=0  RCX1=1.02796280922059  REX1=-0.45202516851367  REX2=-0.47304886171176  RHX1=0.000233272373115809  QSX1=-0.00788307788961443  QSX2=0.954629515459396  QSX3=0.0155855777667025  QSX4=0.125904607142414  QSX5=1.01110069703963  QSX6=20.1938577118433  QSX7=0.310818120717083  QSX8=-0.0430823751139655  QSX9=0.636494404888216  QSX10=0.142438060591663  QSX11=0.346766530036373  QSX12=0  QSX13=0  QSX14=0  PPMX1=0  PCY1=1.34299950037631  PDY1=0.878267729082195  PDY2=-0.0644597923147385  PDY3=0  PEY1=-0.809776534470972  PEY2=-0.600180598867198  PEY3=0.0991732552633487  PEY4=-6.5577974035573  PEY5=0  PKY1=-15.5714726518315  PKY2=1.73126522291751  PKY3=0.365349873517229  PKY4=1.98176755955416  PKY5=0  PKY6=-0.884005199550313  PKY7=-0.237259727611847  PHY1=-0.00183370557235628  PHY2=0.00346401302716671  PVY1=-0.00675427560163264  PVY2=0.036379218103843  PVY3=-0.163543984089166  PVY4=-0.491003349625726  PPY1=-0.62059646553185  PPY2=-0.0647824842338686  PPY3=-0.164648843290686  PPY4=0.283193909060098  PPY5=0  RBY1=10.7588809173639  RBY2=7.70420065295029  RBY3=3.40283755070691e-06  RBY4=0  RCY1=1.06691874059059  REY1=0.308244924574305  REY2=7.48775032604508e-06  RHY1=0.0118479204960415  RHY2=7.63650177161071e-06  RVY1=0.0560024425050078  RVY2=7.48487127056197e-06  RVY3=0  RVY4=98.4047026517149  RVY5=2.02759273900054  RVY6=15.7623064923347  QSY1=0.00699077564863536  QSY2=0  QSY3=0.00153535478298811  QSY4=8.55710322455322e-05  QSY5=0  QSY6=0  QSY7=0.89443879773793  QSY8=-0.403227641260894  QBZ1=11.666656027484  QBZ2=-1.30355438574485  QBZ3=0  QBZ4=0.177918305399071  QBZ5=-0.162481135068033  QBZ6=0  QBZ9=30.1445534682089  QBZ10=0  QCZ1=1.29026978207574  QDZ1=0.0886972644991399  QDZ2=-0.0058634820161856  QDZ3=0.3805597481383  QDZ4=0  QDZ6=0.00160914918118959  QDZ7=-0.00211036330862154  QDZ8=-0.13921904912557  QDZ9=0.00816585550028243  QDZ10=0  QDZ11=0  QEZ1=-2.19802254534746  QEZ2=1.01850535789165  QEZ3=0  QEZ4=0.278379679112054  QEZ5=-0.548414722765386  QHZ1=0.00148361198869669  QHZ2=0.00202017567585904  QHZ3=0.240316641332066  QHZ4=-0.210114035738085  PPZ1=-0.443927982388615  PPZ2=0  SSZ1=0.00914999585397887  SSZ2=0.0389830656052735  SSZ3=0  SSZ4=0  PDXP1=0.396718274678791  PDXP2=0  PDXP3=0  PKYP1=1.00587060633573  PDYP1=0.40483048923438  PDYP2=0  PDYP3=0  PDYP4=0  PHYP1=0.992731942067188  PHYP2=0.150352945499914  PHYP3=0  PHYP4=-3.98988682633674  PECP1=0.502379254513503  PECP2=0  QDTP1=10.0178654287947  QCRP1=0.200627747200702  QCRP2=0.0995735881599772  QBRP1=0.0997107127960717  QDRP1=1.01432910167423  QDRP2=0  aMode=2
  Terminator{7..13} (7 alike) : Terminator
  Wheels : Outport  VectorParamsAs1DForOutWhenUnconnected=off
  wires:
  lambda/1 -> Combined Slip Wheel 2DOF/10
  Combined Slip Wheel 2DOF/1 -> Wheels/1
  Brake Pressure/1 -> Combined Slip Wheel 2DOF/1
  DriveTorque/1 -> Combined Slip Wheel 2DOF/2
  Vx/1 -> Combined Slip Wheel 2DOF/3
  Camber/1 -> Combined Slip Wheel 2DOF/5
  r/1 -> Combined Slip Wheel 2DOF/6
  Press/1 -> Combined Slip Wheel 2DOF/7
  Gnd/1 -> Combined Slip Wheel 2DOF/8
  FzSusp/1 -> Combined Slip Wheel 2DOF/9
  Combined Slip Wheel 2DOF/2 -> Terminator7/1
  Combined Slip Wheel 2DOF/3 -> Terminator8/1
  Combined Slip Wheel 2DOF/4 -> Terminator9/1
  Combined Slip Wheel 2DOF/5 -> Terminator10/1
  Combined Slip Wheel 2DOF/6 -> Terminator11/1
  Combined Slip Wheel 2DOF/7 -> Terminator12/1
  Combined Slip Wheel 2DOF/8 -> Terminator13/1
  Vy/1 -> Combined Slip Wheel 2DOF/4

== system PassVeh14DOF/Wheels and Tires/VDBS/Veh2Tire/Wheel Angles ==
  steer : Inport
  camber : Inport  Port=2
  Constant3 : Constant  Value=ones(1,4).*0
  Reshape : Reshape  OutputDimensionality=Row vector (2-D)
  Reshape1 : Reshape  OutputDimensionality=Row vector (2-D)
  Reshape2 : Reshape  OutputDimensionality=Row vector (2-D)
  Vector Concatenate3 : Concatenate  NumInputs=3  Mode=Multidimensional array
  Vehicle : Outport  VectorParamsAs1DForOutWhenUnconnected=off
  wires:
  Constant3/1 -> Reshape2/1
  Vector Concatenate3/1 -> Vehicle/1
  Reshape/1 -> Vector Concatenate3/3
  Reshape1/1 -> Vector Concatenate3/1
  camber/1 -> Reshape1/1
  Reshape2/1 -> Vector Concatenate3/2
  steer/1 -> Reshape/1

== system PassVeh14DOF/Wheels and Tires/VDBS/Veh2Tire/Wheel to Body Transform ==
  VelVeh : Inport  Partition=on  PartitionDimension=2  PartitionWidth=1  PartitionOffset=0
  WheelAngles : Inport  Port=2  Partition=on  PartitionDimension=2  PartitionWidth=1  PartitionOffset=0
  Constant : Constant  Value=[pi;0;0]
  Demux1 : Demux  Outputs=3
  Divide1 : Product  Inputs=**  Multiplication=Matrix(*)
  Divide2 : Product  Inputs=**  Multiplication=Matrix(*)
  For Each : ForEach  DisableCoverage=on
  Rotation Angles to Direction Cosine Matrix : sharedtransform/Rotation Angles to Direction Cosine Matrix  rotationOrder=ZYX  aMode=2
  Rotation Angles to Direction Cosine Matrix1 : sharedtransform/Rotation Angles to Direction Cosine Matrix  rotationOrder=ZYX  aMode=2
  Selector : Selector  InputPortWidth=3  IndexOptions=Index vector (dialog)  Indices=[3 2 1]  OutputSizes=1
  Selector1 : Selector  InputPortWidth=3  IndexOptions=Index vector (dialog)  Indices=[3 2 1]  OutputSizes=1
  xdotWheel : Outport  ConcatenationDimension=1  VectorParamsAs1DForOutWhenUnconnected=off
  ydotWheel : Outport  Port=2  ConcatenationDimension=1  VectorParamsAs1DForOutWhenUnconnected=off
  zdotWheel : Outport  Port=3  ConcatenationDimension=1  VectorParamsAs1DForOutWhenUnconnected=off
  wires:
  Divide2/1 -> Demux1/1
  Demux1/1 -> xdotWheel/1
  Demux1/2 -> ydotWheel/1
  Demux1/3 -> zdotWheel/1
  Rotation Angles to Direction Cosine Matrix/1 -> Divide1/1
  VelVeh/1 -> Divide1/2
  WheelAngles/1 -> Selector/1
  Selector/1 -> Rotation Angles to Direction Cosine Matrix/1
  Selector1/1 -> Rotation Angles to Direction Cosine Matrix1/1
  Rotation Angles to Direction Cosine Matrix1/1 -> Divide2/1
  Divide1/1 -> Divide2/2
  Constant/1 -> Selector1/1

== system PassVeh14DOF/Wheels and Tires/VDBS/Tires/Fiala Tires/Fx ==
  In1 : Inport
  In2 : Inport  Port=2
  In3 : Inport  Port=3
  In4 : Inport  Port=4
  Bus Selector{,1..3} (4 alike) : BusSelector  OutputSignals=Fx
  Vector Concatenate : Concatenate  NumInputs=4
  Out1 : Outport  VectorParamsAs1DForOutWhenUnconnected=off
  wires:
  Bus Selector3/1 -> Vector Concatenate/4  "<Fx>"
  Bus Selector2/1 -> Vector Concatenate/3  "<Fx>"
  Bus Selector1/1 -> Vector Concatenate/2  "<Fx>"
  In4/1 -> Bus Selector3/1
  In3/1 -> Bus Selector2/1
  In2/1 -> Bus Selector1/1
  Bus Selector/1 -> Vector Concatenate/1  "<Fx>"
  In1/1 -> Bus Selector/1
  Vector Concatenate/1 -> Out1/1

== system PassVeh14DOF/Wheels and Tires/VDBS/Tires/Fiala Tires/Fy ==
  In1 : Inport
  In2 : Inport  Port=2
  In3 : Inport  Port=3
  In4 : Inport  Port=4
  Bus Selector{,1..3} (4 alike) : BusSelector  OutputSignals=Fy
  Vector Concatenate : Concatenate  NumInputs=4
  Out1 : Outport  VectorParamsAs1DForOutWhenUnconnected=off
  wires:
  Vector Concatenate/1 -> Out1/1
  In1/1 -> Bus Selector/1
  Bus Selector/1 -> Vector Concatenate/1  "<Fy>"
  In2/1 -> Bus Selector1/1
  In3/1 -> Bus Selector2/1
  In4/1 -> Bus Selector3/1
  Bus Selector1/1 -> Vector Concatenate/2  "<Fy>"
  Bus Selector2/1 -> Vector Concatenate/3  "<Fy>"
  Bus Selector3/1 -> Vector Concatenate/4  "<Fy>"

== system PassVeh14DOF/Wheels and Tires/VDBS/Tires/Fiala Tires/Fz ==
  In1 : Inport
  In2 : Inport  Port=2
  In3 : Inport  Port=3
  In4 : Inport  Port=4
  Bus Selector{,1..3} (4 alike) : BusSelector  OutputSignals=Fz
  Vector Concatenate : Concatenate  NumInputs=4
  Out1 : Outport  VectorParamsAs1DForOutWhenUnconnected=off
  wires:
  Vector Concatenate/1 -> Out1/1
  In1/1 -> Bus Selector/1
  Bus Selector/1 -> Vector Concatenate/1  "<Fz>"
  In2/1 -> Bus Selector1/1
  In3/1 -> Bus Selector2/1
  In4/1 -> Bus Selector3/1
  Bus Selector1/1 -> Vector Concatenate/2  "<Fz>"
  Bus Selector2/1 -> Vector Concatenate/3  "<Fz>"
  Bus Selector3/1 -> Vector Concatenate/4  "<Fz>"

== system PassVeh14DOF/Wheels and Tires/VDBS/Tires/Fiala Tires/Mx ==
  In1 : Inport
  In2 : Inport  Port=2
  In3 : Inport  Port=3
  In4 : Inport  Port=4
  Bus Selector{,1..3} (4 alike) : BusSelector  OutputSignals=Mx
  Vector Concatenate : Concatenate  NumInputs=4
  Out1 : Outport  VectorParamsAs1DForOutWhenUnconnected=off
  wires:
  Vector Concatenate/1 -> Out1/1
  In1/1 -> Bus Selector/1
  Bus Selector/1 -> Vector Concatenate/1  "<Mx>"
  In2/1 -> Bus Selector1/1
  In3/1 -> Bus Selector2/1
  In4/1 -> Bus Selector3/1
  Bus Selector1/1 -> Vector Concatenate/2  "<Mx>"
  Bus Selector2/1 -> Vector Concatenate/3  "<Mx>"
  Bus Selector3/1 -> Vector Concatenate/4  "<Mx>"

== system PassVeh14DOF/Wheels and Tires/VDBS/Tires/Fiala Tires/My ==
  In1 : Inport
  In2 : Inport  Port=2
  In3 : Inport  Port=3
  In4 : Inport  Port=4
  Bus Selector{,1..3} (4 alike) : BusSelector  OutputSignals=My
  Vector Concatenate : Concatenate  NumInputs=4
  Out1 : Outport  VectorParamsAs1DForOutWhenUnconnected=off
  wires:
  Bus Selector3/1 -> Vector Concatenate/4  "<My>"
  Bus Selector2/1 -> Vector Concatenate/3  "<My>"
  Bus Selector1/1 -> Vector Concatenate/2  "<My>"
  In4/1 -> Bus Selector3/1
  In3/1 -> Bus Selector2/1
  In2/1 -> Bus Selector1/1
  Bus Selector/1 -> Vector Concatenate/1  "<My>"
  In1/1 -> Bus Selector/1
  Vector Concatenate/1 -> Out1/1

== system PassVeh14DOF/Wheels and Tires/VDBS/Tires/Fiala Tires/Mz ==
  In1 : Inport
  In2 : Inport  Port=2
  In3 : Inport  Port=3
  In4 : Inport  Port=4
  Bus Selector{,1..3} (4 alike) : BusSelector  OutputSignals=Mz
  Vector Concatenate : Concatenate  NumInputs=4
  Out1 : Outport  VectorParamsAs1DForOutWhenUnconnected=off
  wires:
  Bus Selector3/1 -> Vector Concatenate/4  "<Mz>"
  Bus Selector2/1 -> Vector Concatenate/3  "<Mz>"
  Bus Selector1/1 -> Vector Concatenate/2  "<Mz>"
  In4/1 -> Bus Selector3/1
  In3/1 -> Bus Selector2/1
  In2/1 -> Bus Selector1/1
  Bus Selector/1 -> Vector Concatenate/1  "<Mz>"
  In1/1 -> Bus Selector/1
  Vector Concatenate/1 -> Out1/1

== system PassVeh14DOF/Wheels and Tires/VDBS/Tires/Fiala Tires/Re ==
  In1 : Inport
  In2 : Inport  Port=2
  In3 : Inport  Port=3
  In4 : Inport  Port=4
  Bus Selector{,1..3} (4 alike) : BusSelector  OutputSignals=Re
  Vector Concatenate : Concatenate  NumInputs=4
  Out1 : Outport  VectorParamsAs1DForOutWhenUnconnected=off
  wires:
  Vector Concatenate/1 -> Out1/1
  In1/1 -> Bus Selector/1
  Bus Selector/1 -> Vector Concatenate/1  "<Re>"
  In2/1 -> Bus Selector1/1
  In3/1 -> Bus Selector2/1
  In4/1 -> Bus Selector3/1
  Bus Selector1/1 -> Vector Concatenate/2  "<Re>"
  Bus Selector2/1 -> Vector Concatenate/3  "<Re>"
  Bus Selector3/1 -> Vector Concatenate/4  "<Re>"

== system PassVeh14DOF/Wheels and Tires/VDBS/Tires/Fiala Tires/alpha ==
  In1 : Inport
  In2 : Inport  Port=2
  In3 : Inport  Port=3
  In4 : Inport  Port=4
  Bus Selector{,1..3} (4 alike) : BusSelector  OutputSignals=Alpha
  Vector Concatenate : Concatenate  NumInputs=4
  Out1 : Outport  VectorParamsAs1DForOutWhenUnconnected=off
  wires:
  Vector Concatenate/1 -> Out1/1
  In1/1 -> Bus Selector/1
  Bus Selector/1 -> Vector Concatenate/1  "<Alpha>"
  In2/1 -> Bus Selector1/1
  In3/1 -> Bus Selector2/1
  In4/1 -> Bus Selector3/1
  Bus Selector1/1 -> Vector Concatenate/2  "<Alpha>"
  Bus Selector2/1 -> Vector Concatenate/3  "<Alpha>"
  Bus Selector3/1 -> Vector Concatenate/4  "<Alpha>"

== system PassVeh14DOF/Wheels and Tires/VDBS/Tires/Fiala Tires/kappa ==
  In1 : Inport
  In2 : Inport  Port=2
  In3 : Inport  Port=3
  In4 : Inport  Port=4
  Bus Selector{,1..3} (4 alike) : BusSelector  OutputSignals=Kappa
  Vector Concatenate : Concatenate  NumInputs=4
  Out1 : Outport  VectorParamsAs1DForOutWhenUnconnected=off
  wires:
  Bus Selector3/1 -> Vector Concatenate/4  "<Kappa>"
  Bus Selector2/1 -> Vector Concatenate/3  "<Kappa>"
  Bus Selector1/1 -> Vector Concatenate/2  "<Kappa>"
  In4/1 -> Bus Selector3/1
  In3/1 -> Bus Selector2/1
  In2/1 -> Bus Selector1/1
  Bus Selector/1 -> Vector Concatenate/1  "<Kappa>"
  In1/1 -> Bus Selector/1
  Vector Concatenate/1 -> Out1/1

== system PassVeh14DOF/Wheels and Tires/VDBS/Tires/Fiala Tires/omega ==
  In1 : Inport
  In2 : Inport  Port=2
  In3 : Inport  Port=3
  In4 : Inport  Port=4
  Bus Selector{,1..3} (4 alike) : BusSelector  OutputSignals=Omega
  Vector Concatenate : Concatenate  NumInputs=4
  Out1 : Outport  VectorParamsAs1DForOutWhenUnconnected=off
  wires:
  In1/1 -> Bus Selector/1
  Bus Selector/1 -> Vector Concatenate/1  "<Omega>"
  In2/1 -> Bus Selector1/1
  In3/1 -> Bus Selector2/1
  In4/1 -> Bus Selector3/1
  Bus Selector1/1 -> Vector Concatenate/2  "<Omega>"
  Bus Selector2/1 -> Vector Concatenate/3  "<Omega>"
  Bus Selector3/1 -> Vector Concatenate/4  "<Omega>"
  Vector Concatenate/1 -> Out1/1

== system PassVeh14DOF/Wheels and Tires/VDBS/Tires/Fiala Tires/z ==
  In1 : Inport
  In2 : Inport  Port=2
  In3 : Inport  Port=3
  In4 : Inport  Port=4
  Bus Selector{,1..3} (4 alike) : BusSelector  OutputSignals=z
  Vector Concatenate : Concatenate  NumInputs=4
  Out1 : Outport  VectorParamsAs1DForOutWhenUnconnected=off
  wires:
  Bus Selector3/1 -> Vector Concatenate/4  "<z>"
  Bus Selector2/1 -> Vector Concatenate/3  "<z>"
  Bus Selector1/1 -> Vector Concatenate/2  "<z>"
  In4/1 -> Bus Selector3/1
  In3/1 -> Bus Selector2/1
  In2/1 -> Bus Selector1/1
  Bus Selector/1 -> Vector Concatenate/1  "<z>"
  In1/1 -> Bus Selector/1
  Vector Concatenate/1 -> Out1/1

== system PassVeh14DOF/Wheels and Tires/VDBS/Tires/Fiala Tires/zdot ==
  In1 : Inport
  In2 : Inport  Port=2
  In3 : Inport  Port=3
  In4 : Inport  Port=4
  Bus Selector{,1..3} (4 alike) : BusSelector  OutputSignals=zdot
  Vector Concatenate : Concatenate  NumInputs=4
  Out1 : Outport  VectorParamsAs1DForOutWhenUnconnected=off
  wires:
  Vector Concatenate/1 -> Out1/1
  In1/1 -> Bus Selector/1
  Bus Selector/1 -> Vector Concatenate/1  "<zdot>"
  In2/1 -> Bus Selector1/1
  In3/1 -> Bus Selector2/1
  In4/1 -> Bus Selector3/1
  Bus Selector1/1 -> Vector Concatenate/2  "<zdot>"
  Bus Selector2/1 -> Vector Concatenate/3  "<zdot>"
  Bus Selector3/1 -> Vector Concatenate/4  "<zdot>"

== system PassVeh14DOF/Wheels and Tires/VDBS/Tires/MF Tires/Fx ==
  In1 : Inport
  In2 : Inport  Port=2
  In3 : Inport  Port=3
  In4 : Inport  Port=4
  Bus Selector{,1..3} (4 alike) : BusSelector  OutputSignals=Fx
  Vector Concatenate : Concatenate  NumInputs=4
  Out1 : Outport  VectorParamsAs1DForOutWhenUnconnected=off
  wires:
  Bus Selector3/1 -> Vector Concatenate/4  "<Fx>"
  Bus Selector2/1 -> Vector Concatenate/3  "<Fx>"
  Bus Selector1/1 -> Vector Concatenate/2  "<Fx>"
  In4/1 -> Bus Selector3/1
  In3/1 -> Bus Selector2/1
  In2/1 -> Bus Selector1/1
  Bus Selector/1 -> Vector Concatenate/1  "<Fx>"
  In1/1 -> Bus Selector/1
  Vector Concatenate/1 -> Out1/1

== system PassVeh14DOF/Wheels and Tires/VDBS/Tires/MF Tires/Fy ==
  In1 : Inport
  In2 : Inport  Port=2
  In3 : Inport  Port=3
  In4 : Inport  Port=4
  Bus Selector{,1..3} (4 alike) : BusSelector  OutputSignals=Fy
  Vector Concatenate : Concatenate  NumInputs=4
  Out1 : Outport  VectorParamsAs1DForOutWhenUnconnected=off
  wires:
  Vector Concatenate/1 -> Out1/1
  In1/1 -> Bus Selector/1
  Bus Selector/1 -> Vector Concatenate/1  "<Fy>"
  In2/1 -> Bus Selector1/1
  In3/1 -> Bus Selector2/1
  In4/1 -> Bus Selector3/1
  Bus Selector1/1 -> Vector Concatenate/2  "<Fy>"
  Bus Selector2/1 -> Vector Concatenate/3  "<Fy>"
  Bus Selector3/1 -> Vector Concatenate/4  "<Fy>"
